simulink model "controller_auno"  (R2025b)
settings: Solver=FixedStepDiscrete  StartTime=0.0  StopTime=10.0  FixedStep=0.1  RelTol=1e-3  EnableMultiTasking=on
libraries: arduinolib x2, arduinosensorlib x1
settings Model: ExtModeTrigDuration=2  Creator=R  LastModifiedBy=R
settings SolverCC: AutoInsertRateTranBlk=on
settings OptimizationCC: EnhancedBackFolding=on  PassReuseOutputArgsAs=Individual arguments  ZeroExternalMemoryAtStartup=off  ZeroInternalMemoryAtStartup=off  MaxStackSize=64  OptimizeBlockOrder=speed  DifferentSizesBufferReuse=on  OptimizationCustomize=off  EfficientTunableParamExpr=on
settings DebuggingCC: ParameterTunabilityLossMsg=error
settings HardwareCC: ProdBitPerInt=16.0  ProdBitPerPointer=16.0  ProdBitPerSizeT=16.0  ProdBitPerPtrDiffT=16.0  ProdLargestAtomicFloat=None  ProdWordSize=8.0  ProdHWDeviceType=Atmel->AVR  UseEmbeddedCoderFeatures=off  UseSimulinkCoderFeatures=off
settings SFSimCC: MATLABDynamicMemAlloc=off
settings RTWCC: SystemTargetFile=ert.tlc  HardwareBoard=Arduino Uno  TemplateMakefile=ert_default_tmf  Toolchain=Arduino AVR  BuildConfiguration=Faster Runs  Description=Embedded Coder
settings CodeAppCC: ForceParamTrailComments=on  IgnoreCustomStorageClasses=off  OperatorAnnotations=on  SimulinkDataObjDesc=on  SFDataObjDesc=on  InsertBlockDesc=on
settings ERTTargetCC: ExtModeTransport=3.0  ExtModeStaticAlloc=on  ExtModeAutomaticAllocSize=off  ExtModeStaticAllocSize=250.0  ExtModeMexFile=ext_xcp  ExtModeIntrfLevel=Level2 - Open  InlinedParameterPlacement=Hierarchical  SupportContinuousTime=on  SupportNonInlinedSFcns=on  SupportVariableSizeSignals=on

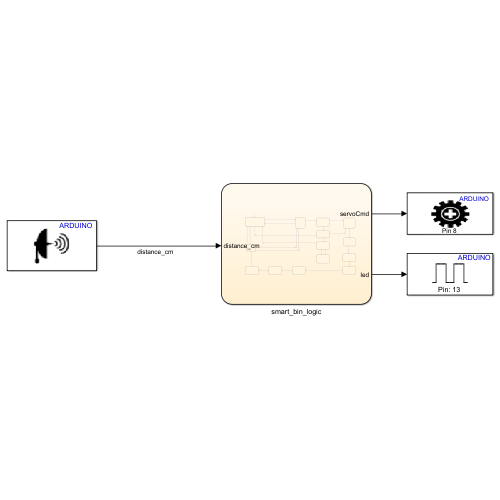
[thumbnail: Simulink's stored preview of the top-level diagram]
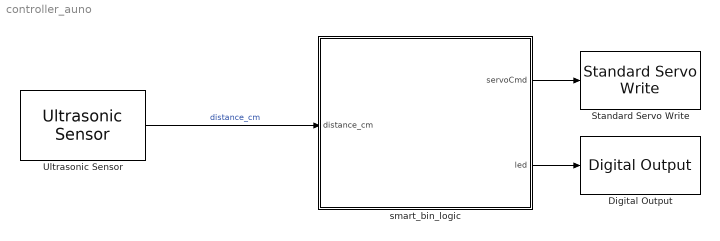
== system controller_auno ==
  Digital Output : arduinolib/Digital Output  pinNumber=13  Direction=output  blockPlatform=arduino
      settings: LibrarySourceBlock=gizmoLibrary/Arduino Utilities/Digital Output
  Standard Servo Write : arduinolib/Standard Servo Write  pinNumber=8  ServoIndex=0  blockPlatform=ARDUINO
  Ultrasonic Sensor : arduinosensorlib/Ultrasonic Sensor  NumSignalPins=2  TrigPin=5  EchoPin=4  SignalPin=3  SampleTime_=0.1  blockPlatform=ARDUINO
  smart_bin_logic : Stateflow chart  TreatAsAtomicUnit=on
  wires:
  Ultrasonic Sensor/1 -> smart_bin_logic/1(distance_cm)  "distance_cm"
  smart_bin_logic/1(servoCmd) -> Standard Servo Write/1
  smart_bin_logic/2(led) -> Digital Output/1

== stateflow chart controller_auno/smart_bin_logic ==
  state CLOSED_IDLE
    entry:
    servoCmd = 0;
    led = 0;
  state REQUEST_WAIT
    entry:
    servoCmd = 0;
    led = 0;
  state HALF_OPEN_BLINK
    entry:
    servoCmd = 90;
    led = 1;
  state OPEN_BLINK
    entry:
    servoCmd = 180;
    led = 1;
  state HALF_OPEN_WAIT
    entry:
    servoCmd = 90;
    led = 0;
  state OPEN_WAIT
    entry:
    servoCmd = 180;
    led = 0;
  state TIMEOUT_BLINK_ON
    entry:
    servoCmd = 0;
    led = 1;
  state TOO_CLOSE
    entry:
    servoCmd = 0;
    led = 1;
  state CLOSE_BLINK1_ON
    entry:
    servoCmd = 0;
    led = 1;
  state TIMEOUT_BLINK_OFF
    entry:
    servoCmd = 0;
    led = 0;
  state COOLDOWN
    entry:
    servoCmd = 0;
    led = 0;
  state CLOSE_BLINK2_OFF
    entry:
    servoCmd = 0;
    led = 0;
  state CLOSE_BLINK2_ON
    entry:
    servoCmd = 0;
    led = 1;
  state CLOSE_BLINK1_OFF
    entry:
    servoCmd = 0;
    led = 0;
  (default) -> CLOSED_IDLE
  CLOSED_IDLE -> REQUEST_WAIT [order 2] : [distance_cm > 0.5 && distance_cm <= 2.5]
  REQUEST_WAIT -> HALF_OPEN_BLINK [order 3] : [after(5, sec)]
  HALF_OPEN_BLINK -> OPEN_BLINK [order 2] : [distance_cm <= 1]
  REQUEST_WAIT -> CLOSED_IDLE [order 1] : [distance_cm > 2.5]
  HALF_OPEN_BLINK -> HALF_OPEN_WAIT [order 1] : [after(1, sec)]
  TOO_CLOSE -> CLOSED_IDLE [order 2] : [distance_cm > 2.5]
  CLOSED_IDLE -> TOO_CLOSE [order 1] : [distance_cm <= 0.5]
  (junction 55) -> CLOSED_IDLE
  (junction 53) -> CLOSED_IDLE
  (junction 49) -> REQUEST_WAIT
  REQUEST_WAIT -> (junction 51) [order 2] : [distance_cm <= 0.5]
  (junction 59) -> OPEN_BLINK
  OPEN_BLINK -> OPEN_WAIT : [after(1, sec)]
  HALF_OPEN_WAIT -> (junction 59) [order 1] : [distance_cm <= 1]
  HALF_OPEN_WAIT -> (junction 55) [order 3] : [distance_cm > 2.5]
  HALF_OPEN_WAIT -> TIMEOUT_BLINK_ON [order 2] : [after(9, sec)]
  TIMEOUT_BLINK_ON -> (junction 53) [order 1] : [distance_cm > 2.5]
  OPEN_WAIT -> CLOSE_BLINK1_ON : [after(9, sec)]
  TOO_CLOSE -> (junction 49) [order 1] : [distance_cm > 0.5 && distance_cm <= 2.5]
  TIMEOUT_BLINK_ON -> TIMEOUT_BLINK_OFF [order 2] : [after(1, sec)]
  TIMEOUT_BLINK_OFF -> TIMEOUT_BLINK_ON : [after(1, sec)]
  (junction 51) -> TOO_CLOSE
  COOLDOWN -> TOO_CLOSE : [after(30, sec)]
  CLOSE_BLINK1_ON -> CLOSE_BLINK1_OFF : [after(1, sec)]
  CLOSE_BLINK2_ON -> CLOSE_BLINK2_OFF : [after(1, sec)]
  CLOSE_BLINK2_OFF -> COOLDOWN : [after(1, sec)]
  CLOSE_BLINK1_OFF -> CLOSE_BLINK2_ON : [after(1, sec)]
  data: distance_cm input; servoCmd output; led output
